simulink model "ADCSSimulator"  (R2024a)
settings: Solver=ode4  StartTime=0.0  StopTime=600  FixedStep=0.01  MaxStep=0.1  RelTol=1e-3  AbsTol=1e-3
values from neighbouring files (symbols this model uses):
  ActuatorAllocationMatrix = ActuatorPhysicalMatrix' * inv(ActuatorPhysicalMatrix * ActuatorPhysicalMatrix')    [set_Init.m]
  ActuatorPhysicalMatrix = [1, 0, 0, 0 ... (first row only)    [set_Init.m]
  albedo_irradiance = 300    [set_Init.m]
  b = 0    [set_Init.m]
  Cd = 2.2    [set_Init.m]
  h_bias = [0; 0; 0]    [set_Init.m]
  J = 4.0e-3 / 628    (= 6.36942675159e-06)    [set_Init.m]
  k_Bdot = ((4 * pi * 0.5236 * 0.0055) / (5677.2 * (4.5e-5)^2))    (= 3147.8423197)    [set_Init.m]
  K_E = K_T    (= 0.0022)    [set_Init.m]
  K_T = 0.0022    [set_Init.m]
  P0 = blkdiag(P0_att, P0_bias)    [set_Init.m]
  P0_att = eye(3) * initial_variance_rad2    [set_Init.m]
  PowerVoltageBus_01 = 3.3    [set_Init.m]
  PowerVoltageBus_02 = 3.3    [set_Init.m]
  PowerVoltageBus_03 = 3.3    [set_Init.m]
  PowerVoltageBus_04 = 3.3    [set_Init.m]
  PowerVoltageBus_05 = 3.3    [set_Init.m]
  PowerVoltageBus_06 = 3.3    [set_Init.m]
  PowerVoltageBus_07 = 3.3    [set_Init.m]
  PowerVoltageBus_08 = 3.3    [set_Init.m]
  PowerVoltageBus_09 = 3.3    [set_Init.m]
  PowerVoltageBus_10 = 3.3    [set_Init.m]
  PowerVoltageBus_11 = 3.3    [set_Init.m]
  PowerVoltageBus_12 = 0.0    (= 0)    [set_Init.m]
  PowerVoltageBus_13 = 0.0    (= 0)    [set_Init.m]
  PowerVoltageBus_14 = 0.0    (= 0)    [set_Init.m]
  PowerVoltageBus_15 = 0.0    (= 0)    [set_Init.m]
  R = 2.0    (= 2)    [set_Init.m]
  ressidual_m = [3e-4; -2e-4; 1e-4]    [set_Init.m]
  solar_irradiance = 1361    [set_Init.m]
  surface_areas = [A_xy, A_yz, A_xz, A_xy, A_yz, A_xz]    [set_Init.m]
  surface_normals_body = [eye(3) -eye(3)]    [set_Init.m]
  surface_positions_body = [       hx,   0,   0 ... (first row only)    [set_Init.m]
  surface_reflectivities = [0.9 0.8 0.9 0.9 0.9 0.9]    [set_Init.m]
  Switch_01 = 1    [set_Init.m]
  Switch_02 = 1    [set_Init.m]
  Switch_03 = 1    [set_Init.m]
  Switch_04 = 1    [set_Init.m]
  Switch_05 = 1    [set_Init.m]
  Switch_06 = 1    [set_Init.m]
  Switch_07 = 1    [set_Init.m]
  Switch_08 = 1    [set_Init.m]
  Switch_09 = 1    [set_Init.m]
  Switch_10 = 1    [set_Init.m]
  Switch_11 = 1    [set_Init.m]
  Switch_12 = 0    [set_Init.m]
  Switch_13 = 0    [set_Init.m]
  Switch_14 = 0    [set_Init.m]
  Switch_15 = 0    [set_Init.m]
  visSampleTime = 0.1    [set_Init.m]
undefined symbols (not defined in the file or in its folder): attitude, Controller, epoch, IAU, juliandate, Kd, km, Kp, m, rad, s, satellite, SGP4_parameters, simulator, UKF_parameters, WMM2020
libraries: sharedtransform x27, aerolibutil x22, aerolibconvert2 x18, simulink_extras x16, matrix_library x6, aerolibtransform2 x4, vrlib x2, aerolibgravity2 x2, aerolibobsolete x1, aerolibattitudesys x1, simulink x1
(part 6 of 8)

== matlab function ADCSSimulator/ADCS/Environment Model/Disturbance Calculator/Solar Radiation Pressure (SRP)/MATLAB Function1 ==
  data: earth_vector_body input; albedo_RP_torque output; surface_normals_body input; surface_areas input; surface_reflectivities input; surface_positions_body input; albedo_irradiance input; albedo_direction_body input
function albedo_RP_torque = Albedo( ...
    earth_vector_body, ...
    surface_normals_body, ...
    surface_areas, ...
    surface_reflectivities, ...
    surface_positions_body, ...
    albedo_irradiance, ...
    albedo_direction_body)
% ALBEDO Calculates torque due to Earth's albedo radiation pressure
%
% Inputs:
%   earth_vector_body         : [3x1] Vector from satellite to Earth center (body frame)
%   surface_normals_body      : [3x6] Normal vectors of each satellite face (body frame)
%   surface_areas             : [1x6] Area of each surface [m^2]
%   surface_reflectivities    : [1x6] Reflectivity coefficient (0 to 1)
%   surface_positions_body    : [3x6] Position vectors from CoM to surface centers [m]
%   albedo_irradiance         : [scalar] Irradiance due to albedo [W/m^2]
%   albedo_direction_body     : [3x1] Direction of incoming albedo light (optional)
%
% Output:
%   albedo_RP_torque          : [3x1] Torque due to albedo radiation pressure [Nm]

% Constants
c = 299792458;                         % Speed of light [m/s]
P = albedo_irradiance / c;            % Radiation pressure [Pa]

% Default albedo direction if not provided
if nargin < 7 || isempty(albedo_direction_body)
    S_albedo = -earth_vector_body / norm(earth_vector_body);  % from Earth to satellite
else
    S_albedo = albedo_direction_body / norm(albedo_direction_body);
end

% Initialize force matrix
F_albedo = zeros(3, 6);

% Loop over each surface
for i = 1:6
    n_i = surface_normals_body(:, i);
    r_i = surface_positions_body(:, i);
    A_i = surface_areas(i);
    R_i = surface_reflectivities(i);

    dot_proj = dot(n_i, S_albedo);

    if dot_proj > 0
        % Force magnitude
        F_mag = -P * A_i * dot_proj;

        % Directional terms
        F_dir = (1 - R_i) * S_albedo + ...
                R_i * (2 * dot_proj * n_i + (2/3) * n_i);

        % Total force vector
        F_albedo(:, i) = F_mag * F_dir;
    end
end

% Compute torque for each face
torques = cross(surface_positions_body, F_albedo, 1);
albedo_RP_torque = sum(torques, 2);

end

== matlab function ADCSSimulator/ADCS/Environment Model/Disturbance Calculator/Solar Radiation Pressure (SRP)/MATLAB Function2 ==
  data: earth_vector_body input; albedo_direction_body output
function albedo_direction_body = fcn(earth_vector_body)
% direction from which the Earth's reflected sunlight (albedo) hits satellite, expressed as a unit vector in the body frame.
albedo_direction_body = -earth_vector_body / norm(earth_vector_body);
end

== matlab function ADCSSimulator/ADCS/Environment Model/Reference Frames Transformations Manager/MATLAB Function ==
  data: r input; SemiMajorAxis output; v input; mu input; Eccentricity output; Inclination output; RightAscension output; ArgumentOfPerigee output; TrueAnomaly output; TrueLongitude output; ArgumentOfLatitude output; LongitudeOfPeriapsis output; SemilatusRectum output; OrbOmega output
%----------------------- Begin Code Sequence -----------------------------%
% Purpose:                                                                %
% Convert a given set of state vectors in ECI reference frame to orbital  %
% elements.                                                               %
%-------------------------------------------------------------------------%
%                                                                         %
% Inputs:                                                                 %
%--------                                                                  
%r_ECI                  [3 x N]                         Position Vector in
%                                                       ECI coordinate
%                                                       frame of reference
%
%v_ECI                  [3 x N]                         Velocity vector in
%                                                       ECI coordinate
%                                                       frame of reference
%
%mu                     double                          Gravitational Constant
%                                                       Defaults to Earth if
%                                                       not specified
% Outputs:
%---------                                                                %
%a                      [1 x N]                         Semi-Major Axis
%                                                       (m)
%
%eMag                   [1 x N]                         Eccentricity
%                                                       (unitless)
%
%i                      [1 x N]                         inclination
%                                                       (rad)
%
%O                      [1 x N]                         Right Ascention of
%                                                       the ascending node
%                                                       (rad)
%
%o                      [1 x N]                         Argument of perigee
%                                                       (rad)
%
%M                      [1 x N]                         Mean Anomaly
%                                                       (rad)
%
%truLon                 [1 x N]                         True Longitude
%                                                       (rad)
%
%argLat                 [1 x N]                         Argument of Latitude
%                                                       (rad)
%
%lonPer                 [1 x N]                         Longitude of Periapse
%                                                       (rad)
%
%p                      [1 x N]                         Semilatus Rectum
%                                                       (m)
%
%OrbOmega                                               Orbital Frame
%                                                       angular velocity
%                                                       (rad)
% References:
%-------------
%Vallado,D. Fundamentals of Astrodynamics and Applications. 2007.
%
% Function Dependencies:
%------------------
%None
%------------------------------------------------------------------       %
% Programed by Darin Koblick  03-04-2012                                  %
% modified by A.H.Khodabakhsh 10-01-2021                                  %
% Updated to address circular equatorial orbits       12/12/2013          %
%------------------------------------------------------------------       %
function [SemiMajorAxis,Eccentricity,Inclination,RightAscension,ArgumentOfPerigee,TrueAnomaly,...
          TrueLongitude,ArgumentOfLatitude,LongitudeOfPeriapsis,SemilatusRectum,OrbOmega] = ...
          StateVector2KeplerianOrbitalElemets(r,v,mu)
% if ~exist('mu','var');  t = getConst(); mu = t.Earth.Mu; end
%Specific angular momentum
h = cross(r,v);
n = cross(repmat([0;0;1],[1,size(r,2)]),h); nMag = sqrt(sum(n.^2,1));
vMag = sqrt(sum(v.^2,1)); 
rMag = sqrt(sum(r.^2,1)); 
hMag = sqrt(sum(h.^2,1));
e = (1./mu).*(bsxfun(@times,(vMag.^2 - mu./rMag),r) - bsxfun(@times,dot(r,v),v)); 
Eccentricity = sqrt(sum(e.^2,1));
zeta = (vMag.^2)./2 - mu./rMag;
%Special Procedure when we have a parabolic orbit
idx = Eccentricity ~= 1;
SemiMajorAxis = zeros(size(Eccentricity));
SemilatusRectum = zeros(size(Eccentricity));
if any(idx)
    SemiMajorAxis(idx) = -mu./(2.*zeta(idx)); 
    SemilatusRectum(idx) = SemiMajorAxis(idx).*(1-Eccentricity(idx).^2); 
else
    SemiMajorAxis(idx) = Inf; 
    SemilatusRectum(idx) = (hMag(idx).^2)./mu; 
end
%Compute the angles
Inclination             = acos(double(single(   h(3,:)./hMag)                   )); 
RightAscension          = acos(double(single(   n(1,:)./nMag)                   ));
ArgumentOfPerigee       = acos(double(single(   dot(n,e)./(nMag.*Eccentricity)) ));
TrueAnomaly             = acos(double(single(   dot(e,r)./(Eccentricity.*rMag)) ));
LongitudeOfPeriapsis    = acos(double(single(   e(1,:)./Eccentricity)           ));
ArgumentOfLatitude      = acos(double(single(   dot(n,r)./(nMag.*rMag))         ));
TrueLongitude           = acos(double(single(   r(1,:)./rMag)                   ));
%Account for those cases where satellite is in circular orbit
         RightAscension   (  n(1,:) == 0) = 0;
       ArgumentOfPerigee  (dot(n,e) == 0) = 0;
      LongitudeOfPeriapsis(  e(1,:) == 0) = 0;
          TrueAnomaly     (dot(e,r) == 0) = 0;
       ArgumentOfLatitude (dot(n,r) == 0) = 0;
%Apply Quadrant Checks to All Determined Angles
idx = n(2,:) < 0; if any(idx),  RightAscension(idx) = 2*pi - RightAscension(idx);  end;
idx = e(3,:) < 0; if any(idx), ArgumentOfPerigee(idx) = 2*pi - ArgumentOfPerigee(idx); end;
idx = dot(r,v) < 0; if any(idx), TrueAnomaly(idx) = 2*pi - TrueAnomaly(idx); end;
idx = e(2,:) < 0; if any(idx), LongitudeOfPeriapsis(idx) = 2*pi-LongitudeOfPeriapsis(idx);  end;
idx = r(3,:) < 0; if any(idx), ArgumentOfLatitude(idx) = 2*pi - ArgumentOfLatitude(idx); end;
idx = r(2,:) < 0; if any(idx), TrueLongitude(idx) = 2*pi - TrueLongitude(idx); end;

rv = zeros(3,1);
rv(:)=cross(r,v); norm_r = norm(r);
OrbOmega = [0;
            dot(v,cross(r./norm_r,rv./norm(rv)))/norm_r;
            0];

% % convert radians to degrees
% r2d = @(x) x.*(180./pi);
% Inclination          = r2d(Inclination         );
% RightAscension       = r2d(RightAscension      );
% ArgumentOfPerigee    = r2d(ArgumentOfPerigee   );
% TrueAnomaly          = r2d(TrueAnomaly         );
% TrueLongitude        = r2d(TrueLongitude       );
% ArgumentOfLatitude   = r2d(ArgumentOfLatitude  );
% LongitudeOfPeriapsis = r2d(LongitudeOfPeriapsis);
% OrbOmega             = r2d(OrbOmega            );
end

== matlab function ADCSSimulator/ADCS/ADCS Hardware/Sensors/Analog Magnetometer Model/MATLAB Function ==
  data: u input; y output
function y = ZeroAvoid(u)
if u ==0
    y = [0.000000001; 0.000000001; 0.000000001];
else
    y = u;
end

== matlab function ADCSSimulator/ADCS/ADCS Hardware/Sensors/Sun Sensor Model/Output NaN in Eclipse ==
  data: u input; y output
function y = replaceZeroWithNaN(u)
%#codegen
    if all(u == 0)
        y = NaN(size(u));
    else
        y = u;
    end
end

== matlab function ADCSSimulator/ADCS/ADCS Software/Attitude Determination/Attitude Estimation Algorithm (MEKF)/MATLAB Function16 ==
  data: q_est output; P_est output; q_feedback input; P_feedback input; P0 input; gyro_meas input; b_sun input; b_mag input; r_sun input; r_mag input; dt input; Q_d input; R_sun input; R_mag input
function [q_est, P_est] = attitude_mekf_robust( ...
    q_feedback, P_feedback, P0, ...
    gyro_meas, b_sun, b_mag, r_sun, r_mag, ...
    dt, Q_d, R_sun, R_mag)
% ATTITUDE_MEKF_ROBUST (Radian-State, Batch-Update, Collinearity-Guarded)
%
% This is a robust MEKF that estimates attitude using a batch update. It
% includes a critical safety check to prevent instability when sensor
% measurement vectors are collinear.
%
% --- UNIT CONVENTION ---
% You must provide inputs in the specified units.
%
% REQUIRED INPUT UNITS:
%   gyro_meas:  Angular velocity [radians/sec, rad/s]
%   P_feedback: Previous error covariance [rad^2]
%   P0:         Initial error covariance  [rad^2]
%   Q_d:        Discrete process noise cov. [rad^2] (Note: Q_d = Qc * dt)
%
%   R_sun:      Sun sensor noise covariance     [unitless^2, for a unit vector]
%   R_mag:      Magnetometer noise covariance   [microTesla^2, µT^2]
%   b_mag:      Magnetic field measurement      [microTesla, µT]
%
% OUTPUT UNITS:
%   q_est:      Estimated attitude quaternion   [unitless]
%   P_est:      Estimated error covariance      [rad^2]
% =========================================================================

% =========================================================================
% 0) INITIALIZATION
% =========================================================================
is_first_run = (norm(q_feedback) < 1e-6);

if is_first_run
    % On the first run, initialize with a default attitude and P0.
    q_prev = [1; 0; 0; 0];
    P_prev = P0;
else
    % Continue propagating the filter's own estimate.
    q_prev = q_feedback;
    P_prev = P_feedback;
end

% =========================================================================
% 1) PREDICTION
% =========================================================================
omega_rad_s = gyro_meas;
q_pred = propagate_with_gyro_expmap(q_prev, omega_rad_s, dt);

% State is 3x1 (d_theta_rad), so Fx is 3x3.
Fx = -skew_symmetric(omega_rad_s);
F = expm(Fx * dt);

% Add the discrete process noise Q_d directly.
P_pred = F * P_prev * F' + Q_d;
P_pred = 0.5 * (P_pred + P_pred'); % Enforce symmetry

% =========================================================================
% 2) BATCH UPDATE
% =========================================================================
% Default the final estimate to the predicted estimate. This will be the
% output if the measurement update is skipped due to collinearity.
q_est = q_pred;
P_est = P_pred;

% --- SAFETY CHECK FOR SENSOR COLLINEARITY ---
perform_update = true; % Assume we will perform an update by default
is_sun_available = ~any(isnan(b_sun));
is_mag_available = ~any(isnan(b_mag));

% Only check for collinearity if both sensors are available for a batch update
if is_sun_available && is_mag_available
    % Define a safety threshold (e.g., skip update if angle < 10 degrees)
    COLLINEARITY_THRESHOLD_DEG = 10.0;
    collinearity_limit = cosd(COLLINEARITY_THRESHOLD_DEG);

    % Calculate the dot product of the two reference vectors.
    r_sun_norm = r_sun / norm(r_sun);
    r_mag_norm = r_mag / norm(r_mag);
    dot_product = abs(dot(r_sun_norm, r_mag_norm));

    if dot_product > collinearity_limit
        perform_update = false;
        fprintf('Warning: Sensor vectors are collinear (angle < %.1f deg). Skipping update.\n', COLLINEARITY_THRESHOLD_DEG);
    end
end

% --- PERFORM BATCH UPDATE ONLY IF SAFE ---
if perform_update
    H_stack = zeros(6,3);
    y_stack = zeros(6,1);
    R_stack = zeros(6,6);
    num_valid_sensors = 0;
    C_pred = quat2rotm(q_pred');

    if is_sun_available
        num_valid_sensors = num_valid_sensors + 1;
        idx = 1:3;
        b_pred_sun = C_pred * r_sun;
        y_sun      = b_sun - b_pred_sun;
        H_sun      = skew_symmetric(b_pred_sun);
        H_stack(idx,:)   = H_sun;
        y_stack(idx)     = y_sun;
        R_stack(idx,idx) = R_sun;
    end

    if is_mag_available
        num_valid_sensors = num_valid_sensors + 1;
        idx = (num_valid_sensors-1)*3 + (1:3);
        b_pred_mag = C_pred * r_mag;
        y_mag      = b_mag - b_pred_mag;
        H_mag      = skew_symmetric(b_pred_mag);
        H_stack(idx,:)   = H_mag;
        y_stack(idx)     = y_mag;
        R_stack(idx,idx) = R_mag;
    end

    if num_valid_sensors > 0
        m = num_valid_sensors * 3;
        H = H_stack(1:m,:);
        y = y_stack(1:m,:);
        R = R_stack(1:m,1:m);

        S = H*P_pred*H' + R;
        S = 0.5*(S + S');

        K = (P_pred*H') / S;
        dtheta_rad = K * y;
        dq = [1; 0.5*dtheta_rad];
        dq = dq / norm(dq);
        
        % Overwrite the predicted state with the updated state
        q_est = quat_multiply(q_pred, dq);

        I_KH = eye(3) - K*H;
        P_est = I_KH*P_pred*I_KH' + K*R*K';
        P_est = 0.5*(P_est + P_est');
    end
end

% =========================================================================
% 3) FINALIZATION
% =========================================================================
% Final normalization and sign convention for uniqueness.
q_est = q_est / norm(q_est);
% if q_est(1) < 0
%     q_est = -q_est; % Enforce positive scalar part
% end
% 
end

% =========================================================================
% HELPER FUNCTIONS
% =========================================================================
function q_out = propagate_with_gyro_expmap(q_prev, omega_rad_s, dt)
    theta = norm(omega_rad_s) * dt;
    if theta > 1e-9
        axis = omega_rad_s / (theta/dt);
        dq = [cos(0.5*theta); axis * sin(0.5*theta)];
        q_out = quat_multiply(q_prev, dq);
    else
        q_out = q_prev;
    end
    q_out = q_out / norm(q_out);
end

function C = skew_symmetric(v)
    C = [  0   -v(3)  v(2);
          v(3)   0   -v(1);
         -v(2)  v(1)   0  ];
end

function q_out = quat_multiply(q1, q2)
    w1 = q1(1); v1 = q1(2:4);
    w2 = q2(1); v2 = q2(2:4);
    w  = w1*w2 - dot(v1,v2);
    v  = w1*v2 + w2*v1 + cross(v1,v2);
    q_out = [w; v];
end

== matlab function ADCSSimulator/ADCS/ADCS Software/Attitude Determination/Attitude Estimation Algorithm (MEKF)/MATLAB Function17 ==
  data: q_est output; P_est output; q_feedback input; P_feedback input; q_quest input; gyro_meas input; b_sun input; b_mag input; r_sun input; r_mag input; dt input; Q_noise input; R_sun input; R_mag input; time input; P0 input
function [q_est, P_est] = attitude_mekf( ...
    q_feedback, P_feedback, ...
    q_quest, ...
    gyro_meas, b_sun, b_mag, r_sun, r_mag, ...
    dt, Q_noise, R_sun, R_mag, time, P0)
% ATTITUDE_EKF_SIMPLIFIED (Quaternion Estimation Only)
%
% This is a simplified, robust MEKF that only estimates the attitude.
% It uses a safe initialization and robustly hybridizes with QUEST
% solutions when they are available and of high quality.
%
% --- UNIT CONVENTION ---
% Attitude Error State & Covariance: milli-radians (rad)
% Gyro Measurement:                radians/second (rad/s)
% Magnetic Field Measurement:      micro-Tesla (uT)
%
% Sun Sensor Noise R_sun:          radians^2 (rad^2)
% Mag Sensor Noise R_mag:          micro-Tesla^2 (uT^2)
% Process Noise Q_noise (3x3):     (rad/s)^2
% =========================================================================
% 0) INITIALIZATION & HYBRIDIZATION
% =========================================================================
is_sun_available = ~any(isnan(b_sun));
is_quest_valid = is_sun_available && ~any(isnan(q_quest));

% Check if this is the first run of the simulation
is_first_run = (norm(q_feedback) < 1e-6);

if is_first_run
    % On the first run, ALWAYS initialize with a default attitude and
    % a very large uncertainty to ensure a safe start.
    q_prev = [1;0;0;0];
    P_prev = P0; % Huge uncertainty
else
    % --- Standard Operation: Check for Reset ---
    perform_reset = false;
    if is_quest_valid

        if time == 3
            perform_reset = true;
        end
    end

    if perform_reset
        % Reset the state using the high-quality QUEST solution
        q_prev = q_quest;
        P_prev = eye(3) * (1.0 * (pi/180))^2;
    else
        % No reset, continue propagating the filter's own estimate
        q_prev = q_feedback;
        P_prev = P_feedback;
    end
end

% =========================================================================
% 1) PREDICTION
% =========================================================================
omega = gyro_meas; % No bias estimation
q_pred = propagate_with_gyro_expmap(q_prev, omega, dt);

% State is 3x1 (d_theta), so Fx is 3x3
Fx = -skew_symmetric(omega);
F = expm(Fx * dt);

P_pred = F * P_prev * F' + Q_noise;
P_pred = 0.5 * (P_pred + P_pred'); % Enforce symmetry

% =========================================================================
% 2) BATCH UPDATE
% =========================================================================
q_est = q_pred;
P_est = P_pred;

H_stack = zeros(6,3);
y_stack = zeros(6,1);
R_stack = zeros(6,6);
num_valid = 0;
C_pred = quat2rotm(q_pred');

% --- Sun Sensor Measurement
if is_sun_available
    num_valid = num_valid + 1;
    idx = 1:3;
    b_pred_sun = C_pred * r_sun;
    y_sun      = b_sun - b_pred_sun;
    H_sun      = skew_symmetric(b_pred_sun);

    H_stack(idx,:) = H_sun;
    y_stack(idx)   = y_sun;
    R_stack(idx,idx) = R_sun;
end

% --- Magnetometer Measurement ---
if ~any(isnan(b_mag))
    num_valid = num_valid + 1;
    idx = (num_valid-1)*3 + (1:3);
    b_pred_mag = C_pred * r_mag;
    y_mag      = b_mag - b_pred_mag;
    H_mag      = skew_symmetric(b_pred_mag);

    H_stack(idx,:)   = H_mag;
    y_stack(idx)     = y_mag;
    R_stack(idx,idx) = R_mag;
end

% --- Perform Update ---
if num_valid > 0
    m = num_valid*3;
    H = H_stack(1:m,:);
    y = y_stack(1:m,:);
    R = R_stack(1:m,1:m);

    S = H*P_pred*H' + R;
    S = 0.5*(S + S');

    K = (P_pred*H') / S;

    dtheta_mrad = K * y;
    dtheta_rad = dtheta_mrad;

    dq = [1; 0.5*dtheta_rad];
    dq = dq / norm(dq);

    q_est = quat_multiply(q_pred, dq);

    I_KH = eye(3) - K*H;
    P_est = I_KH*P_pred*I_KH' + K*R*K';
    P_est = 0.5*(P_est + P_est');
end

q_est = q_est / norm(q_est);

end

% =========================================================================
% Helper Functions
% =========================================================================
function q_out = propagate_with_gyro_expmap(q_prev, omega_rad_s, dt)
    theta = norm(omega_rad_s) * dt;
    if theta > 1e-9
        axis = omega_rad_s / (theta/dt);
        half = 0.5*theta;
        dq = [cos(half); axis * sin(half)];
        q_out = quat_multiply(q_prev, dq);
    else
        q_out = q_prev;
    end
    q_out = q_out / norm(q_out);
end

function C = skew_symmetric(v)
    C = [   0   -v(3)  v(2);
          v(3)    0   -v(1);
         -v(2)  v(1)    0  ];
end

function q_out = quat_multiply(q1, q2)
    w1 = q1(1); v1 = q1(2:4);
    w2 = q2(1); v2 = q2(2:4);
    w  = w1*w2 - dot(v1,v2);
    v  = w1*v2 + w2*v1 + cross(v1,v2);
    q_out = [w; v];
end

== matlab function ADCSSimulator/ADCS/ADCS Software/Attitude Determination/Attitude Estimation Algorithm (MEKF)/MATLAB Function18 ==
  data: q_est output; P_est output; q_feedback input; b_feedback input; P_feedback input; P0 input; gyro_meas input; b_sun input; b_mag input; r_sun input; r_mag input; dt input; Q_v input; Q_u input; R_sun input; R_mag input; b_est output; y_out output; A output
function [q_est, P_est, b_est, y_out, A] = attitude_mekf_robust_6state( ...
    q_feedback, b_feedback, P_feedback, P0, ...
    gyro_meas, b_sun, b_mag, r_sun, r_mag, ...
    dt, Q_v, Q_u, R_sun, R_mag)
% This function implements a robust, 6-state MEKF to estimate both attitude
% (quaternion) and gyroscope bias. It uses a consistent right-multiplicative
% error-state formulation and a proper sequential update for measurements.

% =========================================================================
% 0) INITIALIZATION
% =========================================================================
% On the first run, P_feedback can be empty or zero.
% if isempty(P_feedback) || norm(P_feedback) == 0
%     P_minus = P0;
%     b_minus = b_feedback; % initial guess for bias
%     q_minus = [1; 0; 0; 0]; % Default to identity quaternion
% else
%     P_minus = P_feedback;
%     b_minus = b_feedback;
%     q_minus = q_feedback;
% end
P_minus = P_feedback;
b_minus = b_feedback;
q_minus = q_feedback;
% Always normalize the input quaternion for stability
q_minus = q_minus / norm(q_minus);

% =========================================================================
% 1) PREDICTION (PROPAGATION)
% =========================================================================
% Compensate gyro measurement with the current bias estimate
omega = gyro_meas - b_minus;

% Quaternion Propagation (Right-Multiplication)
theta_vec = omega * dt;
phi = norm(theta_vec);
if phi == 0
    % No rotation, delta quaternion is identity
    q_delta = [1; 0; 0; 0];
else
    axis = theta_vec / phi;
    q_delta = [cos(phi / 2); sin(phi / 2) * axis];
end
% CORRECTED: Apply rotation in the body frame (Right Multiplication)
q_propagated = quat_mult(q_minus, q_delta);
q_propagated = q_propagated / norm(q_propagated);

% Covariance Propagation
skew_omega = cross_matrix(omega);
F = [-skew_omega, -eye(3); ...
     zeros(3,3), zeros(3,3)];

% IMPROVED: Using matrix exponential for higher accuracy
Phi = expm(F * dt);

% Discretize continuous noise matrices Q_v and Q_u
Qd = blkdiag(Q_v, Q_u) * dt;
P_propagated = Phi * P_minus * Phi' + Qd;
P_propagated = 0.5 * (P_propagated + P_propagated'); % Enforce symmetry

% =========================================================================
% 2) SEQUENTIAL MEASUREMENT UPDATE
% =========================================================================
% Initialize estimates with propagated values. These will be updated by
% the available sensor measurements sequentially.
q_updated = q_propagated;
b_updated = b_minus;
P_updated = P_propagated;

% First Update: Sun Sensor
sun_available = (norm(b_sun) > 1e-6) && (norm(r_sun) > 1e-6);
y_out = NaN(3,1);
A = NaN(3,3);
if sun_available
    A = quat_to_dcm(q_updated);
    h_sun = A * r_sun;
    y_sun = b_sun - h_sun;
    y_out = y_sun;
    H_sun = [cross_matrix(h_sun), zeros(3,3)];

    S_sun = H_sun * P_updated * H_sun' + R_sun;
    K_sun = (P_updated * H_sun') / S_sun;
    delta_x = K_sun * y_sun;

    delta_a = delta_x(1:3); % Attitude error component
    delta_b = delta_x(4:6); % Bias error component

    % Correct the state
    delta_q = [1; 0.5 * delta_a];
    delta_q = delta_q / norm(delta_q);
    q_updated = quat_mult(q_updated, delta_q);
    b_updated = b_updated + delta_b;

    % Update covariance using the robust Joseph form
    IKH = eye(6) - K_sun * H_sun;
    P_updated = IKH * P_updated * IKH' + K_sun * R_sun * K_sun';
    P_updated = 0.5 * (P_updated + P_updated');
end

% Second Update: Magnetometer
% mag_available = (norm(b_mag) > 1e-6) && (norm(r_mag) > 1e-6);
% y_out = NaN(3,1);
% if mag_available
%     % Use the state updated by the sun sensor (if available)
%     A = quat_to_dcm(q_updated);
%     h_mag = A * r_mag;
%     y_mag = b_mag - h_mag;
%     y_out = y_mag;
%     H_mag = [cross_matrix(h_mag), zeros(3,3)];
% 
%     % Use the covariance updated by the sun sensor
%     S_mag = H_mag * P_updated * H_mag' + R_mag;
%     K_mag = (P_updated * H_mag') / S_mag;
%     delta_x = K_mag * y_mag;
% 
%     delta_a = delta_x(1:3);
%     delta_b = delta_x(4:6);
% 
%     % Correct the state again
%     delta_q = [1; 0.5 * delta_a];
%     delta_q = delta_q / norm(delta_q);
%     q_updated = quat_mult(q_updated, delta_q);
%     b_updated = b_updated + delta_b;
% 
%     % Update covariance again
%     IKH = eye(6) - K_mag * H_mag;
%     P_updated = IKH * P_updated * IKH' + K_mag * R_mag * K_mag';
%     P_updated = 0.5 * (P_updated + P_updated');
% end

% =========================================================================
% 3) FINAL OUTPUT
% =========================================================================
q_est = q_updated / norm(q_updated);
P_est = P_updated;
b_est = b_updated;
% Enforce sign convention for uniqueness (positive scalar)
if q_est(1) < 0
    q_est = -q_est;
end

end

% =========================================================================
% HELPER FUNCTIONS (Updated for [scalar; vector] convention)
% =========================================================================
function C = cross_matrix(v)
    % Creates a skew-symmetric cross-product matrix from a 3x1 vector
    C = [  0   -v(3)  v(2);
          v(3)   0   -v(1);
         -v(2)  v(1)   0  ];
end

function r = quat_mult(q1, q2)
    % Performs quaternion multiplication for q = [w; x; y; z]
    w1 = q1(1); v1 = q1(2:4);
    w2 = q2(1); v2 = q2(2:4);
    
    w = w1*w2 - dot(v1, v2);
    v = w1*v2 + w2*v1 + cross(v1, v2);
    r = [w; v];
end

function A = quat_to_dcm(q)
    % Converts a quaternion q = [w; x; y; z] to a DCM
    w = q(1); v = q(2:4);
    
    skew_v = cross_matrix(v);
    A = eye(3) + 2*w*skew_v + 2*skew_v*skew_v;
end

== matlab function ADCSSimulator/ADCS/ADCS Software/Attitude Determination/Attitude Estimation Algorithm (MEKF)/Ensure Quaternion Continuity1/Ensure Quaternion Continuity ==
  data: q_new input; q_out output; q_prev input
function q_out = quaternion_continuity(q_new, q_prev)
%%%%%%%%%%%%%%%%%%%%%%%%%%%%%%%%%%%%%%%%%%%%%%%%%%%%%%%%%%%%%%%%%%%%%%%%
%   QUATERNION_CONTINUITY Ensures continuous quaternion output.
%
%   q_out = ensure_quaternion_continuity(q_new, q_prev) selects between
%   q_new and -q_new to ensure the shortest rotational path from q_prev,
%   preventing sign-flipping discontinuities in simulations.
%
%   Inputs:
%       q_new   - 4x1 newly calculated quaternion. Can be in either
%                 scalar-first or scalar-last format.
%       q_prev  - 4x1 quaternion from the previous time step. Must be in
%                 the same format as q_new.
%
%   Output:
%       q_out   - The 4x1 quaternion (either q_new or -q_new) that is
%                 mathematically closer to q_prev.
%%%%%%%%%%%%%%%%%%%%%%%%%%%%%%%%%%%%%%%%%%%%%%%%%%%%%%%%%%%%%%%%%%%%%%%%

    % 1. Input Validation (optional for Simulink if types are enforced)
    % coder.extrinsic('error'); % Uncomment if you need error checking
    % if ~isequal(size(q_new), [4,1]) || ~isequal(size(q_prev), [4,1])
    %     error('Input quaternions must be 4x1 column vectors.');
    % end

    % 2. Calculate the Euclidean distance (norm) to both possible rotations
    % The quaternions q and -q represent the same physical rotation. We want
    % to choose the one that is numerically closer to the previous state to
    % avoid a "jump" in the data when plotted.
    dist_to_positive_q = norm(q_new - q_prev);
    dist_to_negative_q = norm(-q_new - q_prev);

    % 3. Select the quaternion on the shortest path
    if dist_to_negative_q < dist_to_positive_q
        q_out = -q_new;
    else
        q_out = q_new;
    end
end

== matlab function ADCSSimulator/ADCS/ADCS Software/Attitude Determination/Attitude Estimation Algorithm (MEKF)/MATLAB Function19 ==
  data: p input; trace_p output
function trace_p = Trace(p)

trace_p = trace(p);

== matlab function ADCSSimulator/ADCS/ADCS Software/Attitude Determination/Attitude Estimation Algorithm (MEKF)/MATLAB Function20 ==
  data: q_est output; P_est output; q_feedback input; P_feedback input; gyro_meas input; b_mag input; r_mag input; dt input; Q_noise input; R_mag input; P0 input
function [q_est, P_est] = attitude_mekf_diagnostic( ...
    q_feedback, P_feedback, ...
    gyro_meas, b_mag, r_mag, ...
    dt, Q_noise, R_mag, P0)
% ATTITUDE_EKF_DIAGNOSTIC (Magnetometer-Only Test)
%
% This is a special diagnostic version of the MEKF that ONLY uses the
% magnetometer. It does not use the gyroscope or sun sensor. Its sole

% purpose is to verify the correctness of the magnetometer data path.
%
% --- UNIT CONVENTION ---
% Attitude Error State & Covariance: milli-radians (mrad)
% Magnetic Field Measurement:      micro-Tesla (uT)
%
% Mag Sensor Noise R_mag:          micro-Tesla^2 (uT^2)
% Process Noise Q_noise (3x3):     (mrad)^2
% =========================================================================
% 0) INITIALIZATION & STATE SELECTION
% =========================================================================
is_first_run = (norm(q_feedback) < 1e-6);

if is_first_run
    % On the first run, initialize with a default attitude.
    q_prev = [1; 0; 0; 0];
    P_prev = P0; % Use the P0 from your tuning script
else
    % Propagate from the previous state
    q_prev = q_feedback;
    P_prev = P_feedback;
end

% =========================================================================
% 1) PREDICTION (GYRO IS IGNORED)
% =========================================================================
% For this test, we assume no motion between steps. The prediction is just
% the previous state plus a small amount of process noise.
q_pred = q_prev;
P_pred = P_prev + Q_noise; % Add process noise
P_pred = 0.5 * (P_pred + P_pred'); % Enforce symmetry

% =========================================================================
% 2) UPDATE (MAGNETOMETER ONLY)
% =========================================================================
q_est = q_pred;
P_est = P_pred;

% --- Perform Update if Magnetometer is Available ---
if ~any(isnan(b_mag))
    C_pred = quat2rotm(q_pred');
    
    b_pred_mag = C_pred * r_mag;
    y_mag      = b_mag - b_pred_mag;
    H_mag      = skew_symmetric(b_pred_mag) / 1000; % Maps d(theta)_mrad to d(y)_uT

    S = H_mag*P_pred*H_mag' + R_mag;
    S = 0.5*(S + S');
    
    K = (P_pred*H_mag') / S;
    
    dtheta_mrad = K * y_mag;
    dtheta_rad = dtheta_mrad / 1000;
    
    dq = [1; 0.5*dtheta_rad];
    dq = dq / norm(dq);
    
    q_est = quat_multiply(q_pred, dq);
    
    I_KH = eye(3) - K*H_mag;
    P_est = I_KH*P_pred*I_KH' + K*R_mag*K';
    P_est = 0.5*(P_est + P_est');
end

q_est = q_est / norm(q_est);

end

% =========================================================================
% Helper Functions
% =========================================================================
function C = skew_symmetric(v)
    C = [   0   -v(3)  v(2);
          v(3)    0   -v(1);
         -v(2)  v(1)    0  ];
end

function q_out = quat_multiply(q1, q2)
    w1 = q1(1); v1 = q1(2:4);
    w2 = q2(1); v2 = q2(2:4);
    w  = w1*w2 - dot(v1,v2);
    v  = w1*v2 + w2*v1 + cross(v1,v2);
    q_out = [w; v];
end

== matlab function ADCSSimulator/ADCS/ADCS Software/Attitude Determination/Attitude Estimation Algorithm (MEKF)/Quaternion Error (deg)2 ==
  data: q_true input; error_angle_deg output; q_est input
function error_angle_deg = quaternion_angle_error(q_true, q_est)
% Calculates the angular error between two quaternions

% Inputs:
%   q_true: 4x1 true attitude quaternion [scalar; vector].
%   q_est:  4x1 estimated attitude quaternion [scalar; vector].
%
% Output:
%   error: 180-deg error.

    % Validate input dimensions.
    if ~isequal(size(q_true), [4,1]) || ~isequal(size(q_est), [4,1])
        error('Input quaternions must be 4x1 column vectors.');
    end
error_angle_deg = 2 * acos(abs(dot(q_true, q_est))) * 180 / pi;
   
end

== matlab function ADCSSimulator/ADCS/ADCS Software/MATLAB Function1 ==
  data: current_error input; rmse_out output
function rmse_out = fcn(current_error)
%#codegen

% تعریف متغیرهای پایدار برای ذخیره مقادیر بین گام‌های زمانی
% sum_sq_error: مجموع مربع خطاها تا این لحظه
% count: تعداد نمونه‌ها (گام‌های زمانی) تا این لحظه
persistent sum_sq_error count;

% --- مقداردهی اولیه در اولین اجرای شبیه‌سازی ---
% این شرط فقط در اولین گام زمانی (t=0) اجرا می‌شود
if isempty(sum_sq_error)
    sum_sq_error = 0;
    count = 0;
end

% --- به‌روزرسانی در هر گام زمانی ---
% 1. تعداد نمونه‌ها را یکی اضافه کن
count = count + 1;

% 2. مربع خطای ورودی فعلی را به مجموع کل اضافه کن
sum_sq_error = sum_sq_error + current_error^2;

% 3. میانگین مربعات خطا (MSE) را محاسبه کن
mean_sq_error = sum_sq_error / count;

% 4. جذر آن را برای به دست آوردن RMSE محاسبه کن
rmse_out = sqrt(mean_sq_error);

end

== matlab function ADCSSimulator/ADCS/ADCS Software/Onboard Calendar/Clock Synchronizer ==
  data: onboard_rtc_julian_date input; corrected_julian_date_utc output; gps_julian_date input; is_gps_time_valid input; dt input; drift_correction_sec output
function [corrected_julian_date_utc, drift_correction_sec] = synchronize_onboard_clock(onboard_rtc_julian_date, gps_julian_date, is_gps_time_valid, dt)
% synchronize_onboard_clock Corrects the onboard clock using GPS time.
%
% Function Objective:
% This function implements the core logic for synchronizing a satellite's
% onboard Real-Time Clock (RTC) with a high-accuracy time source from a GPS
% receiver. This is a critical task to prevent time drift in the flight software.
%
% Inputs:
%   onboard_rtc_julian_date: (double) The current time from the satellite's
%                                     internal, free-running clock.
%   gps_julian_date:         (double) The high-accuracy time provided by the
%                                     GPS receiver for the current moment.
%   is_gps_time_valid:       (logical) A flag (true/false) indicating if the
%                                     GPS receiver has a valid time lock.
%   dt:                      (double) The time step of the simulation or software
%                                     cycle, in seconds.
%
% Outputs:
%   corrected_julian_date_utc: (double) The new, corrected Julian Date that should
%                                       be used to set the onboard RTC.
%   drift_correction_sec:      (double) The magnitude of the correction that was just
%                                       applied, in seconds. This is useful for
%                                       telemetry and health monitoring.

    % Default Output Initialization
    % Assume no correction will be made initially.
    drift_correction_sec = 0.0;
    
    % --- Main Synchronization Logic ---
    % Check if we have a valid time signal from the GPS receiver.
    if is_gps_time_valid
        % GPS Time is VALID: Perform Correction
        % The GPS time is considered the absolute "truth".
        
        % Calculate the drift between the onboard clock and the GPS time.
        % The difference is in days, so we multiply by 86400 to get seconds.
        drift_correction_sec = (onboard_rtc_julian_date - gps_julian_date) * 86400.0;
        
        % The new, corrected time is simply the GPS time. The flight
        % software would now use this value to command the RTC hardware
        % to reset itself.
        corrected_julian_date_utc = gps_julian_date;
        
    else
        % GPS Time is INVALID: Propagate Onboard Time
        % If there's no valid GPS signal, we cannot correct the clock.
        % We must trust our onboard RTC and let it continue to run.
        
        % We propagate the onboard clock forward by one time step (dt).
        % We convert dt from seconds to days for the Julian Date calculation.
        corrected_julian_date_utc = onboard_rtc_julian_date + (dt / 86400.0);
    end
end

== matlab function ADCSSimulator/ADCS/ADCS Software/Onboard Calendar/JD to Decimal Year ==
  data: jd input; dec_year output
function dec_year = jd_to_decimal_year(jd)
% jd_to_decimal_year Converts a Julian Date to a decimal year.
%
% Inputs:
%   jd: (double) The Julian Date to be converted.
%
% Output:
%   dec_year: (double) The date as a decimal year (e.g., 2025.5).

    % Convert Julian date to a standard calendar date vector
    date_vec = datevec(datetime(jd, 'ConvertFrom', 'juliandate'));
    year = date_vec(1);
    
    % Find the Julian date for the start of the current year (Jan 1, 00:00)
    jd_start_of_year = juliandate(datetime(year, 1, 1, 0, 0, 0));
    
    % Find the Julian date for the start of the next year
    jd_start_of_next_year = juliandate(datetime(year + 1, 1, 1, 0, 0, 0));
    
    % Calculate the total number of days in the current year
    days_in_year = jd_start_of_next_year - jd_start_of_year;
    
    % Calculate the number of days (including fractional part) that have passed
    % in the current year.
    days_passed = jd - jd_start_of_year;
    
    % The decimal year is the base year plus the fraction of the year that has passed.
    dec_year = year + (days_passed / days_in_year);

end

== stateflow chart ADCSSimulator/ADCS/ADCS Software/Attitude Control/Chart ==
  settings: sampleTime=0.1
  state Off
  state Transition
    SysMode;
  state Detumbling
  state Nadir_Pointing
  state Sun_Pointing
  Transition -> Off [order 4] : [SysMode == 0]
  (default) -> Transition
  Transition -> Detumbling [order 2] : [SysMode == 1]
  Transition -> Nadir_Pointing [order 1] : [SysMode == 2]
  Transition -> Sun_Pointing [order 3] : [SysMode == 3]
  data: sf_internal_action_state_placeholder_data local double size=1 =0; sf_internal_action_state_placeholder_data local double size=1 =0; sf_internal_action_state_placeholder_data local double size=1 =0; sf_internal_action_state_placeholder_data local double size=1 =0; SysMode input; MeasuredMagneticField_Body input; TorqueCommand output; DipoleCommand output; MeasuredAngularVelocity_Body input; ICRF2BodyQuaternions input; qDesired_NadirPointing input; qDesired_SunPointing input; ErrorQuaternion output; Wheel_Momentum_Vector input

== matlab function ADCSSimulator/ADCS/ADCS Software/Attitude Control/Chart/Nadir_Pointing/َAttitude Controller (LQR Controller)/LQR Quaternion Feedback Controller/Torque to Dipole Converter ==
  data: B_body input; torque_cmd_body input; dipole_cmd_body output
function dipole_cmd_body = calculateMTQDipole(B_body, torque_cmd_body)
% calculateMTQDipole Converts a commanded torque to a commanded dipole moment.
%
% This function takes the desired torque from a controller and the local
% magnetic field vector to calculate the required magnetic dipole moment
% for the magnetorquers (MTQs).
%
% It inherently handles the physical limitation that torque cannot be
% generated parallel to the magnetic field.
%
% Inputs:
%   tau_cmd_body: 3x1 vector of the commanded torque in the body frame (N*m)
%   B_body:       3x1 vector of the magnetic field in the body frame (Tesla)
%
% Output:
%   m_cmd_body:   3x1 vector of the commanded magnetic dipole moment (A*m^2)

    % Calculate the squared magnitude of the magnetic field
    B_sq = dot(B_body, B_body);

    % Prevent division by zero if the magnetic field is negligible
    if B_sq < 1e-12 % (equivalent to a field of 1 nT)
        dipole_cmd_body = [0; 0; 0];
        return;
    end
    
    % Calculate the required dipole moment.
    % The formula m = cross(B, tau) / ||B||^2 finds the dipole that
    % generates the component of tau perpendicular to B. The component of
    % tau parallel to B is automatically ignored by the cross product.
    dipole_cmd_body = cross(B_body, torque_cmd_body) / B_sq;

end

== matlab function ADCSSimulator/ADCS/ADCS Software/Attitude Control/Chart/Sun_Pointing/Sun Pointing Algorithm (LQR)/LQR Quaternion Feedback Controller/Torque to Dipole Converter ==
  data: B_body input; torque_cmd_body input; dipole_cmd_body output
function dipole_cmd_body = calculateMTQDipole(B_body, torque_cmd_body)
% calculateMTQDipole Converts a commanded torque to a commanded dipole moment.
%
% This function takes the desired torque from a controller and the local
% magnetic field vector to calculate the required magnetic dipole moment
% for the magnetorquers (MTQs).
%
% It inherently handles the physical limitation that torque cannot be
% generated parallel to the magnetic field.
%
% Inputs:
%   tau_cmd_body: 3x1 vector of the commanded torque in the body frame (N*m)
%   B_body:       3x1 vector of the magnetic field in the body frame (Tesla)
%
% Output:
%   m_cmd_body:   3x1 vector of the commanded magnetic dipole moment (A*m^2)

    % Calculate the squared magnitude of the magnetic field
    B_sq = dot(B_body, B_body);

    % Prevent division by zero if the magnetic field is negligible
    if B_sq < 1e-12 % (equivalent to a field of 1 nT)
        dipole_cmd_body = [0; 0; 0];
        return;
    end
    
    % Calculate the required dipole moment.
    % The formula m = cross(B, tau) / ||B||^2 finds the dipole that
    % generates the component of tau perpendicular to B. The component of
    % tau parallel to B is automatically ignored by the cross product.
    dipole_cmd_body = cross(B_body, torque_cmd_body) / B_sq;

end

== matlab function ADCSSimulator/ADCS/ADCS Software/Attitude Control/Chart/Sun_Pointing/Sun Pointing Algorithm (PD)/PD Quaternion Feedback Controller/Torque to Dipole Converter ==
  data: B_body input; torque_cmd_body input; dipole_cmd_body output
function dipole_cmd_body = calculateMTQDipole(B_body, torque_cmd_body)
% calculateMTQDipole Converts a commanded torque to a commanded dipole moment.
%
% This function takes the desired torque from a controller and the local
% magnetic field vector to calculate the required magnetic dipole moment
% for the magnetorquers (MTQs).
%
% It inherently handles the physical limitation that torque cannot be
% generated parallel to the magnetic field.
%
% Inputs:
%   tau_cmd_body: 3x1 vector of the commanded torque in the body frame (N*m)
%   B_body:       3x1 vector of the magnetic field in the body frame (Tesla)
%
% Output:
%   m_cmd_body:   3x1 vector of the commanded magnetic dipole moment (A*m^2)

    % Calculate the squared magnitude of the magnetic field
    B_sq = dot(B_body, B_body);

    % Prevent division by zero if the magnetic field is negligible
    if B_sq < 1e-12 % (equivalent to a field of 1 nT)
        dipole_cmd_body = [0; 0; 0];
        return;
    end
    
    % Calculate the required dipole moment.
    % The formula m = cross(B, tau) / ||B||^2 finds the dipole that
    % generates the component of tau perpendicular to B. The component of
    % tau parallel to B is automatically ignored by the cross product.
    dipole_cmd_body = cross(B_body, torque_cmd_body) / B_sq;

end

== matlab function ADCSSimulator/ADCS/ADCS Software/Onboard Reference Frames Transformations Manager1/Ensure Quaternion Continuity/Ensure Quaternion Continuity ==
  data: q_new input; q_out output; q_prev input
function q_out = quaternion_continuity(q_new, q_prev)
%%%%%%%%%%%%%%%%%%%%%%%%%%%%%%%%%%%%%%%%%%%%%%%%%%%%%%%%%%%%%%%%%%%%%%%%
%   QUATERNION_CONTINUITY Ensures continuous quaternion output.
%
%   q_out = ensure_quaternion_continuity(q_new, q_prev) selects between
%   q_new and -q_new to ensure the shortest rotational path from q_prev,
%   preventing sign-flipping discontinuities in simulations.
%
%   Inputs:
%       q_new   - 4x1 newly calculated quaternion. Can be in either
%                 scalar-first or scalar-last format.
%       q_prev  - 4x1 quaternion from the previous time step. Must be in
%                 the same format as q_new.
%
%   Output:
%       q_out   - The 4x1 quaternion (either q_new or -q_new) that is
%                 mathematically closer to q_prev.
%%%%%%%%%%%%%%%%%%%%%%%%%%%%%%%%%%%%%%%%%%%%%%%%%%%%%%%%%%%%%%%%%%%%%%%%

    % 1. Input Validation (optional for Simulink if types are enforced)
    % coder.extrinsic('error'); % Uncomment if you need error checking
    % if ~isequal(size(q_new), [4,1]) || ~isequal(size(q_prev), [4,1])
    %     error('Input quaternions must be 4x1 column vectors.');
    % end

    % 2. Calculate the Euclidean distance (norm) to both possible rotations
    % The quaternions q and -q represent the same physical rotation. We want
    % to choose the one that is numerically closer to the previous state to
    % avoid a "jump" in the data when plotted.
    dist_to_positive_q = norm(q_new - q_prev);
    dist_to_negative_q = norm(-q_new - q_prev);

    % 3. Select the quaternion on the shortest path
    if dist_to_negative_q < dist_to_positive_q
        q_out = -q_new;
    else
        q_out = q_new;
    end
end
